simulink model "AGV_IFOC_BLOCKS"  (R2025a)
settings: Solver=ode4  StartTime=0.0  StopTime=t_stop_agv  FixedStep=h_step_agv  RelTol=1e-3
InitFcn:
  | addpath(fileparts(get_param('AGV_IFOC_BLOCKS','FileName'))); bm_drive = 'IFOC'; bm_model = 'AGV_IFOC_BLOCKS'; block_model_params;
values from neighbouring files (symbols this model uses):
  agv_fault_side_default = a.fault_side    [block_model_params.m]
  agv_fault_type_default = a.fault_type    [block_model_params.m]
  Bm = m.B    [block_model_params.m]
  Crr = a.Crr    [block_model_params.m]
  Esw = P.inv.Esw    [block_model_params.m]
  eta_g = a.eta_g    [block_model_params.m]
  flux_mode_default = c.flux_mode    [block_model_params.m]
  G_gear = a.G    [block_model_params.m]
  h_step_agv = 25e-6    (= 2.5e-05)    [block_model_params.m]
  Iref_sw = P.inv.Iref    [block_model_params.m]
  Jm = m.J    [block_model_params.m]
  ke = m.ke    [block_model_params.m]
  kh = m.kh    [block_model_params.m]
  Ki_i = c.Ki_i    [block_model_params.m]
  Ko = c.Ko    [block_model_params.m]
  Kp_i = c.Kp_i    [block_model_params.m]
  Kp_w = c.Kp_w    [block_model_params.m]
  L_look = a.L_look    [block_model_params.m]
  Llr = m.Llr    [block_model_params.m]
  Lls = m.Lls    [block_model_params.m]
  Lm0 = m.Lm0    [block_model_params.m]
  Lm_rated = m.Lm_rated    [block_model_params.m]
  lut_an = P.lut.psi    [block_model_params.m]
  lut_ml = bm_P.lut.psi; end    [block_model_params.m]
  lut_T = P.lut.T(:)'    [block_model_params.m]
  lut_w = P.lut.w(:)'    [block_model_params.m]
  Lx = a.Lx    [block_model_params.m]
  Ly = a.Ly    [block_model_params.m]
  m_payload = a.m_payload    [block_model_params.m]
  m_robot = a.m_robot    [block_model_params.m]
  mlp_b1 = double(bm_M.b1(:))    [block_model_params.m]
  mlp_b2 = double(bm_M.b2)    [block_model_params.m]
  mlp_W1 = double(bm_M.W1)    [block_model_params.m]
  mlp_W2 = double(bm_M.W2(:)')    [block_model_params.m]
  mlp_x_mu = double(bm_M.x_mu(:))    [block_model_params.m]
  mlp_x_sd = double(bm_M.x_sd(:))    [block_model_params.m]
  mlp_y_mu = double(bm_M.y_mu)    [block_model_params.m]
  mlp_y_sd = double(bm_M.y_sd)    [block_model_params.m]
  mras_Ki = c.mras_Ki    [block_model_params.m]
  mras_Kp = c.mras_Kp    [block_model_params.m]
  mras_wc = c.mras_wc    [block_model_params.m]
  NT_agv = max(1, round(Ts/h_step_agv))    [block_model_params.m]
  pp = m.p    [block_model_params.m]
  psi_k = m.psi_k    [block_model_params.m]
  r_wheel = a.r_wheel    [block_model_params.m]
  rce = P.inv.rce    [block_model_params.m]
  Rr = m.Rr    [block_model_params.m]
  Rs = m.Rs    [block_model_params.m]
  s32 = sqrt(3)/2    [block_model_params.m]
  sat_a = m.sat_a    [block_model_params.m]
  sat_b = m.sat_b    [block_model_params.m]
  sat_on = m.sat_on    [block_model_params.m]
  Te_max = c.Te_max    [block_model_params.m]
  Ts = P.ctrl.Ts    [block_log_to_thesis.m]    (also in block_model_params.m = c.Ts)
  twopi = 2*pi    (= 6.28318530718)    [block_model_params.m]
  Vce0 = P.inv.Vce0    [block_model_params.m]
  Vdc = P.inv.Vdc    [block_model_params.m]
  Vref_sw = P.inv.Vref    [block_model_params.m]
  W_track = a.W_track    [block_model_params.m]
(part 1 of 4)
settings Model: Creator=ironman  LastModifiedBy=ironman
settings DataIOCC: SaveOutput=off  SignalLogging=off  SaveTime=off

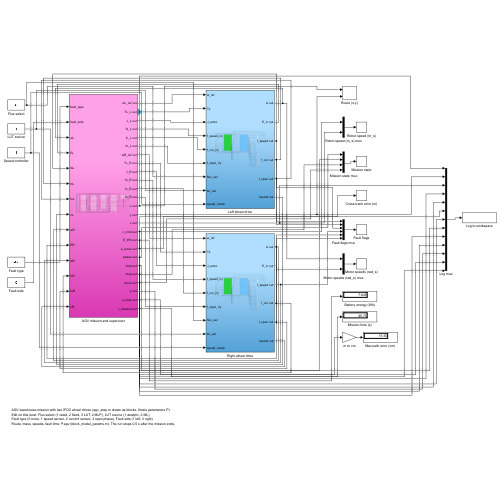
[thumbnail: Simulink's stored preview of the top-level diagram]
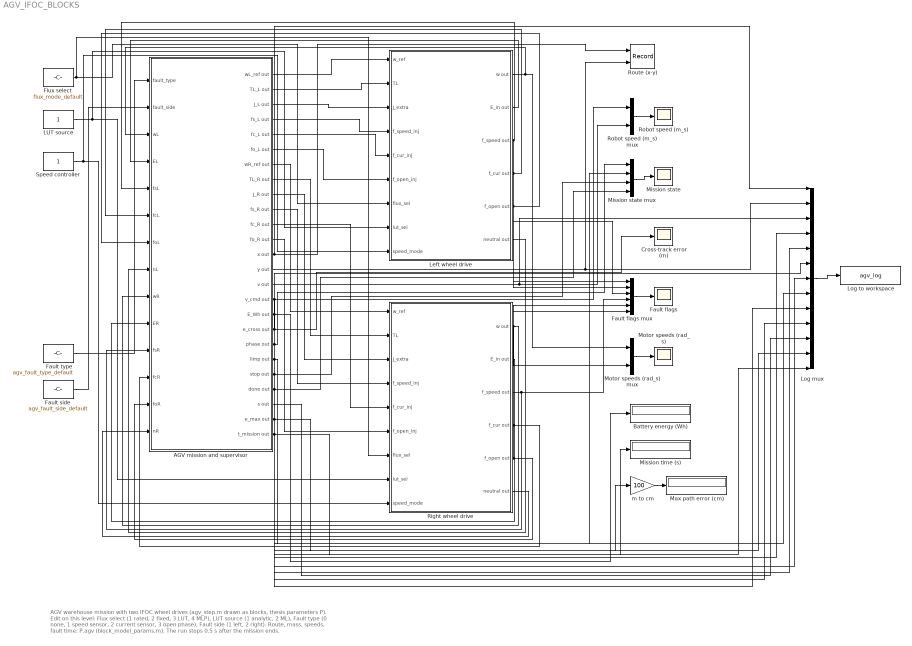
== system AGV_IFOC_BLOCKS ==
  note: AGV warehouse mission with two IFOC wheel drives (agv_step.m drawn as blocks, thesis parameters P).
      | Edit on this level: Flux select (1 rated, 2 fixed, 3 LUT, 4 MLP), LUT source (1 analytic, 2 ML),
      | Fault type (0 none, 1 speed sensor, 2 current sensor, 3 open phase), Fault side (1 left, 2 right).
      | Route, mass, speeds, fault time: P.agv (block_model_params.m). The run stops 0.5 s after the mission ends.
  AGV mission and supervisor : Subsystem
  Battery energy (Wh) : Display
  Cross-track error (m) : Scope
  Fault flags : Scope
  Fault flags mux : Mux  Inputs=6
  Fault side : Constant  Value=agv_fault_side_default
  Fault type : Constant  Value=agv_fault_type_default
  Flux select : Constant  Value=flux_mode_default
  LUT source : Constant
  Left wheel drive : Subsystem
  Log mux : Mux  Inputs=13
  Log to workspace : ToWorkspace  VariableName=agv_log  SaveFormat=Structure With Time  SampleTime=-1
      settings: Decimation=40
  Max path error (cm) : Display
  Mission state : Scope
  Mission state mux : Mux
  Mission time (s) : Display
  Motor speeds (rad_s) : Scope
  Motor speeds (rad_s) mux : Mux  Inputs=2
  Right wheel drive : Subsystem
  Robot speed (m_s) : Scope
  Robot speed (m_s) mux : Mux  Inputs=2
  Route (x-y) : Record  NumPorts=2.0  FileSettingsInternal="{\"entries\":[{\"content\":{\"excelSettings\":{\"content\":{},\"type\":\"Streamout.ExcelSettings\"},\"parquetSettings\":{\"content\":{},\"type\":\"Streamout.ParquetSettings\"}},\"type\":\"Streamout.FileSettingStorage\",\"uuid\":\"\"}],\"packageUris\":[\"http:\\/\\/schema.mathworks.com\\/mf0\\/streamout_blocks\\/R2020a\"],\"version\":\"1.0\"}"  FrameSettings=[0, 0]  Layout=[1 1]  SignalsInternal="{\"entries\":[{\"content\":{\"signals\":[{\"content\":{\"blockPath\":[],\"dimensions\":[1],\"domain\":\"\",\"lineColor\":\"#a2142f\",\"plots\":[ 1 ],\"port\":1,\"sid\":[\"\"],\"signalID\":1,\"signalName\":\"AGV mission and supervisor:13\"},\"type\":\"RecordBlkView.Signal\",\"uuid\":\"\"},{\"content\":{\"blockPath\":[],\"dimensions\":[1],\"domain\":\"\",\"lineColor\":\"#139fff\",\"plots\":[ 1 ],\"port\":2,\"sid\":[\"\"],\"signalID\":2,\"signalName\":\"AGV mission and supervisor:14\"},\"type\":\"RecordBlkView.Signal\",\"uuid\":\"\"}]},\"type\":\"RecordBlkView.InputSignals\",\"uuid\":\"\"}],\"packageUris\":[\"http:\\/\\/schema.mathworks.com\\/mf0\\/streamout_blocks\\/R2020a\"],\"version\":\"1.0\"}"  VisualizationBindings="{\"xyplotplugin\":{\"info\":[{\"series\":[{\"bindingParametersList\":[{\"parameter\":\"X-Axis\",\"signalID\":1,\"signalName\":\"AGV mission and supervisor:13\"},{\"parameter\":\"Y-Axis\",\"signalID\":2,\"signalName\":\"AGV mission and supervisor:14\"}],\"seriesID\":0}],\"subplotID\":1}]}}"  CompatibilityTag=XY
  Speed controller : Constant
  m to cm : Gain  Gain=100
  wires:
  AGV mission and supervisor/1(wL_ref out) -> Left wheel drive/1(w_ref)
  AGV mission and supervisor/2(TL_L out) -> Left wheel drive/2(TL)
  AGV mission and supervisor/3(J_L out) -> Left wheel drive/3(J_extra)
  AGV mission and supervisor/4(fs_L out) -> Left wheel drive/4(f_speed_inj)
  AGV mission and supervisor/5(fc_L out) -> Left wheel drive/5(f_cur_inj)
  AGV mission and supervisor/6(fo_L out) -> Left wheel drive/6(f_open_inj)
  Flux select/1 -> Left wheel drive/7(flux_sel), Right wheel drive/7(flux_sel)
  LUT source/1 -> Left wheel drive/8(lut_sel), Right wheel drive/8(lut_sel)
  Speed controller/1 -> Left wheel drive/9(speed_mode), Right wheel drive/9(speed_mode)
  AGV mission and supervisor/7(wR_ref out) -> Right wheel drive/1(w_ref)
  AGV mission and supervisor/8(TL_R out) -> Right wheel drive/2(TL)
  AGV mission and supervisor/9(J_R out) -> Right wheel drive/3(J_extra)
  AGV mission and supervisor/10(fs_R out) -> Right wheel drive/4(f_speed_inj)
  AGV mission and supervisor/11(fc_R out) -> Right wheel drive/5(f_cur_inj)
  AGV mission and supervisor/12(fo_R out) -> Right wheel drive/6(f_open_inj)
  Fault type/1 -> AGV mission and supervisor/1(fault_type)
  Fault side/1 -> AGV mission and supervisor/2(fault_side)
  Left wheel drive/1(w out) -> AGV mission and supervisor/3(wL), Motor speeds (rad_s) mux/1
  Left wheel drive/2(E_in out) -> AGV mission and supervisor/4(EL)
  Left wheel drive/3(f_speed out) -> AGV mission and supervisor/5(fsL), Fault flags mux/1
  Left wheel drive/4(f_cur out) -> AGV mission and supervisor/6(fcL), Fault flags mux/2
  Left wheel drive/5(f_open out) -> AGV mission and supervisor/7(foL), Fault flags mux/3
  Left wheel drive/6(neutral out) -> AGV mission and supervisor/8(nL)
  Right wheel drive/1(w out) -> AGV mission and supervisor/9(wR), Motor speeds (rad_s) mux/2
  Right wheel drive/2(E_in out) -> AGV mission and supervisor/10(ER)
  Right wheel drive/3(f_speed out) -> AGV mission and supervisor/11(fsR), Fault flags mux/4
  Right wheel drive/4(f_cur out) -> AGV mission and supervisor/12(fcR), Fault flags mux/5
  Right wheel drive/5(f_open out) -> AGV mission and supervisor/13(foR), Fault flags mux/6
  Right wheel drive/6(neutral out) -> AGV mission and supervisor/14(nR)
  AGV mission and supervisor/13(x out) -> Route (x-y)/1, Log mux/1
  AGV mission and supervisor/14(y out) -> Route (x-y)/2, Log mux/2
  AGV mission and supervisor/16(v_cmd out) -> Robot speed (m_s) mux/1, Log mux/4
  AGV mission and supervisor/15(v out) -> Robot speed (m_s) mux/2, Log mux/3
  Robot speed (m_s) mux/1 -> Robot speed (m_s)/1
  AGV mission and supervisor/19(phase out) -> Mission state mux/1, Log mux/7
  AGV mission and supervisor/20(limp out) -> Mission state mux/2, Log mux/8
  AGV mission and supervisor/21(stop out) -> Mission state mux/3, Log mux/9
  AGV mission and supervisor/22(done out) -> Mission state mux/4, Log mux/10
  Mission state mux/1 -> Mission state/1
  AGV mission and supervisor/18(e_cross out) -> Cross-track error (m)/1, Log mux/6
  Fault flags mux/1 -> Fault flags/1
  Motor speeds (rad_s) mux/1 -> Motor speeds (rad_s)/1
  AGV mission and supervisor/17(E_Wh out) -> Battery energy (Wh)/1, Log mux/5
  AGV mission and supervisor/25(t_mission out) -> Mission time (s)/1, Log mux/13
  AGV mission and supervisor/24(e_max out) -> m to cm/1, Log mux/12
  m to cm/1 -> Max path error (cm)/1
  AGV mission and supervisor/23(s out) -> Log mux/11
  Log mux/1 -> Log to workspace/1

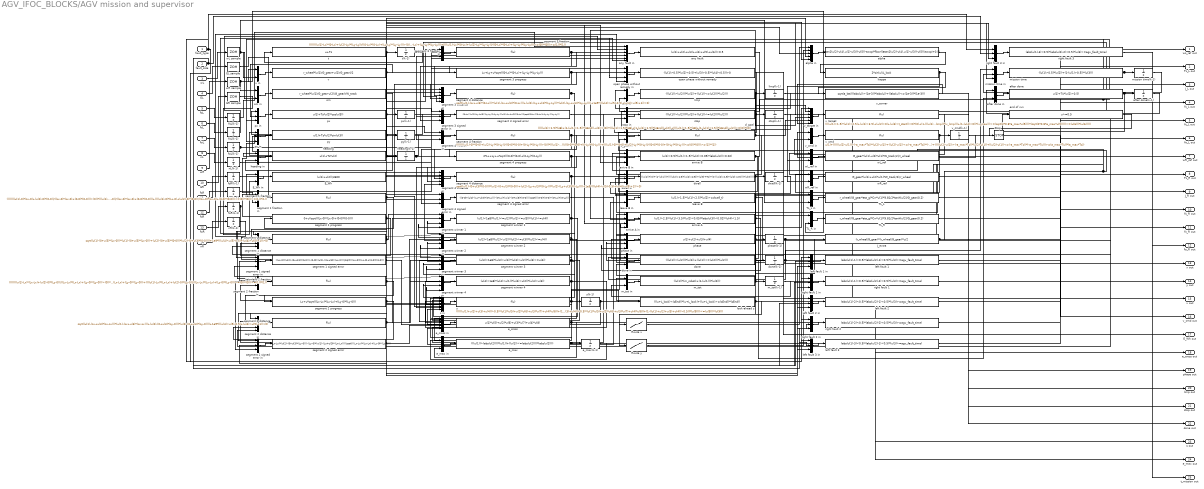
== system AGV_IFOC_BLOCKS/AGV mission and supervisor ==
  fault_type : Inport
  fault_side : Inport  Port=2
  wL : Inport  Port=3
  EL : Inport  Port=4
  fsL : Inport  Port=5
  fcL : Inport  Port=6
  foL : Inport  Port=7
  nL : Inport  Port=8
  wR : Inport  Port=9
  ER : Inport  Port=10
  fsR : Inport  Port=11
  fcR : Inport  Port=12
  foR : Inport  Port=13
  nR : Inport  Port=14
  EL sample : ZeroOrderHold  SampleTime=Ts
  ER sample : ZeroOrderHold  SampleTime=Ts
  E_Wh : Fcn  Expr=(u(1)+u(2))/3600
  E_Wh in : Mux  Inputs=2
  J_extra : Fcn  Expr=(r_wheel/G_gear)*(r_wheel/G_gear)*u/2
  Route x : Lookup_n-D  NumberOfTableDimensions=1  BreakpointsForDimension1=[0 Lx Lx+Ly 2*Lx+Ly 2*(Lx+Ly)]  Table=[0 Lx Lx 0 0]  ExtrapMethod=Clip  InternalRulePriority=Speed  RndMeth=Simplest
  Route y : Lookup_n-D  NumberOfTableDimensions=1  BreakpointsForDimension1=[0 Lx Lx+Ly 2*Lx+Ly 2*(Lx+Ly)]  Table=[0 0 Ly Ly 0]  ExtrapMethod=Clip  InternalRulePriority=Speed  RndMeth=Simplest
  Stop : Stop
  TL_L : Fcn  Expr=r_wheel/(G_gear*eta_g)*Crr*u(1)*9.81/2*tanh(u(2)/G_gear/0.2)
  TL_L in : Mux  Inputs=2
  TL_R : Fcn  Expr=r_wheel/(G_gear*eta_g)*Crr*u(1)*9.81/2*tanh(u(2)/G_gear/0.2)
  TL_R in : Mux  Inputs=2
  after done : Fcn  Expr=u(1)+Ts*(u(2)>0.5)
  after done in : Mux  Inputs=2
  after done(k-1) : UnitDelay  SampleTime=Ts  HasFrameUpgradeWarning=on
  alpha : Fcn  Expr=(atan2(u(2)-u(4),u(1)-u(3))-u(5))-twopi*floor((atan2(u(2)-u(4),u(1)-u(3))-u(5))/twopi+0.5)
  alpha in : Mux  Inputs=5
  any fault : Fcn  Expr=(u(1)+u(2)+u(3)+u(4)+u(5)+u(6))>0.5
  any fault in : Mux  Inputs=6
  arrive A : Fcn  Expr=(u(1)>2.5)*(u(1)<3.5)*(u(2)<0.05)*(abs(u(3))<0.02)*(u(4)<1.5)
  arrive A in : Mux
  arrive B : Fcn  Expr=(u(1)>0.5)*(u(1)<1.5)*(u(2)<0.05)*(abs(u(3))<0.02)
  arrive B in : Mux  Inputs=3
  d_goal : Fcn  Expr=(((((u(1)<1.5)*(sB)+(1-(u(1)<1.5))*(sEnd))-u(2))>(0))*(((u(1)<1.5)*(sB)+(1-(u(1)<1.5))*(sEnd))-u(2))+((((u(1)<1.5)*(sB)+(1-(u(1)<1.5))*(sEnd))-u(2))<=(0))*(0))
  d_goal in : Mux  Inputs=2
  done : Fcn  Expr=(((u(1))>(u(2)))*(u(1))+((u(1))<=(u(2)))*(u(2)))
  done in : Mux  Inputs=2
  done(k-1) : UnitDelay  SampleTime=Ts  HasFrameUpgradeWarning=on
  dwell : Fcn  Expr=((u(1))*(0)+(1-(u(1)))*((((u(2)>1.5)*(u(2)<2.5))*(u(3)+Ts)+(1-((u(2)>1.5)*(u(2)<2.5)))*(u(3)))))
  dwell in : Mux  Inputs=3
  dwell(k-1) : UnitDelay  SampleTime=Ts  HasFrameUpgradeWarning=on
  e_cross : Fcn  Expr=u(1)*u(5)+u(2)*u(6)+u(3)*u(7)+u(4)*u(8)
  e_cross in : Mux  Inputs=8
  e_max : Fcn  Expr=(((u(1))>(abs(u(2))))*(u(1))+((u(1))<=(abs(u(2))))*(abs(u(2))))
  e_max in : Mux  Inputs=2
  e_max(k-1) : UnitDelay  SampleTime=Ts  HasFrameUpgradeWarning=on
  end of run : Fcn  Expr=u>=0.5
  fcL(k-1) : UnitDelay  SampleTime=Ts  HasFrameUpgradeWarning=on
  fcR(k-1) : UnitDelay  SampleTime=Ts  HasFrameUpgradeWarning=on
  foL(k-1) : UnitDelay  SampleTime=Ts  HasFrameUpgradeWarning=on
  foR(k-1) : UnitDelay  SampleTime=Ts  HasFrameUpgradeWarning=on
  fsL(k-1) : UnitDelay  SampleTime=Ts  HasFrameUpgradeWarning=on
  fsR(k-1) : UnitDelay  SampleTime=Ts  HasFrameUpgradeWarning=on
  heading : Fcn  Expr=u(1)+Ts*u(2)
  heading in : Mux  Inputs=2
  heading(k-1) : UnitDelay  SampleTime=Ts  HasFrameUpgradeWarning=on
  kappa : Fcn  Expr=2*sin(u)/L_look
  leave B : Fcn  Expr=(u(1)>1.5)*(u(1)<2.5)*(u(2)>=dwell_t)
  leave B in : Mux  Inputs=2
  left fault 1 : Fcn  Expr=(abs(u(1)-1)<0.5)*(abs(u(2)-1)<0.5)*(u(3)>=agv_fault_time)
  left fault 1 in : Mux  Inputs=3
  left fault 2 : Fcn  Expr=(abs(u(1)-2)<0.5)*(abs(u(2)-1)<0.5)*(u(3)>=agv_fault_time)
  left fault 2 in : Mux  Inputs=3
  left fault 3 : Fcn  Expr=(abs(u(1)-3)<0.5)*(abs(u(2)-1)<0.5)*(u(3)>=agv_fault_time)
  left fault 3 in : Mux  Inputs=3
  limp : Fcn  Expr=(((u(1))>(u(2)))*(u(1))+((u(1))<=(u(2)))*(u(2)))
  limp in : Mux  Inputs=2
  limp(k-1) : UnitDelay  SampleTime=Ts  HasFrameUpgradeWarning=on
  look-ahead s : Fcn  Expr=(((u+L_look)<(sEnd))*(u+L_look)+((u+L_look)>=(sEnd))*(sEnd))
  m_tot : Fcn  Expr=((u(1))*(m_robot)+(1-(u(1)))*(u(2)))
  m_tot in : Mux  Inputs=2
  m_tot(k-1) : UnitDelay  InitialCondition=m_robot+m_payload  SampleTime=Ts  HasFrameUpgradeWarning=on
  mission time : Fcn  Expr=((u(1)>0.5)*(u(2))+(1-(u(1)>0.5))*(u(3)))
  mission time in : Mux  Inputs=3
  mission time(k-1) : UnitDelay  SampleTime=Ts  HasFrameUpgradeWarning=on
  nL(k-1) : UnitDelay  SampleTime=Ts  HasFrameUpgradeWarning=on
  nR(k-1) : UnitDelay  SampleTime=Ts  HasFrameUpgradeWarning=on
  om : Fcn  Expr=r_wheel*(u(1)/G_gear-u(2)/G_gear)/W_track
  om in : Mux  Inputs=2
  open phase without remedy : Fcn  Expr=((u(1)>0.5)*(u(2)<0.5)+(u(3)>0.5)*(u(4)<0.5))>0
  open phase without remedy in : Mux
  phase : Fcn  Expr=u(1)+u(2)+u(3)+u(4)
  phase in : Mux
  phase(k-1) : UnitDelay  InitialCondition=1  SampleTime=Ts  HasFrameUpgradeWarning=on
  px : Fcn  Expr=u(1)+Ts*u(2)*cos(u(3))
  px in : Mux  Inputs=3
  px(k-1) : UnitDelay  SampleTime=Ts  HasFrameUpgradeWarning=on
  py : Fcn  Expr=u(1)+Ts*u(2)*sin(u(3))
  py in : Mux  Inputs=3
  py(k-1) : UnitDelay  SampleTime=Ts  HasFrameUpgradeWarning=on
  right fault 1 : Fcn  Expr=(abs(u(1)-1)<0.5)*(abs(u(2)-2)<0.5)*(u(3)>=agv_fault_time)
  right fault 1 in : Mux  Inputs=3
  right fault 2 : Fcn  Expr=(abs(u(1)-2)<0.5)*(abs(u(2)-2)<0.5)*(u(3)>=agv_fault_time)
  right fault 2 in : Mux  Inputs=3
  right fault 3 : Fcn  Expr=(abs(u(1)-3)<0.5)*(abs(u(2)-2)<0.5)*(u(3)>=agv_fault_time)
  right fault 3 in : Mux  Inputs=3
  s : Fcn  Expr=((((((u(1)+u(2)+u(3)+u(4))>0.5)*(u(1)*u(5)+u(2)*u(6)+u(3)*u(7)+u(4)*u(8))+(1-((u(1)+u(2)+u(3)+u(4))>0.5))*(u(9))))>(u(9)))*((((u(1)+u(2)+u(3)+u(4))>0.5)*(u(1)*u(5)+u(2)*u(6)+u(3)*u(7)+u(4)*u(8))+(1-((u(1)+u(2)+u(3)+u(4))>0.5))*(u(9))))+(((((u(1)+u(2)+u(3)+u(4))>0.5)*(u(1)*u(5)+u(2)*u(6)+u(3)*u(7)+u(4)*u(8))+(1-((u(1)+u(2)+u(3)+u(4))>0.5))*(u(9))))<=(u(9)))*(u(9)))
  s in : Mux  Inputs=9
  s(k-1) : UnitDelay  SampleTime=Ts  HasFrameUpgradeWarning=on
  segment 1 distance : Fcn  Expr=sqrt((u(1)-(0+u(3)*(Lx-0)))*(u(1)-(0+u(3)*(Lx-0)))+(u(2)-(0+u(3)*(0-0)))*(u(2)-(0+u(3)*(0-0))))+1e9*(((u(4)<u(5)-0.5)+(u(4)>u(5)+1))>0)
  segment 1 distance in : Mux  Inputs=5
  segment 1 fraction : Fcn  Expr=((((((((u(1)-0)*(Lx-0)+(u(2)-0)*(0-0))/((Lx-0)*(Lx-0)+(0-0)*(0-0)))>(0))*(((u(1)-0)*(Lx-0)+(u(2)-0)*(0-0))/((Lx-0)*(Lx-0)+(0-0)*(0-0)))+((((u(1)-0)*(Lx-0)+(u(2)-0)*(0-0))/((Lx-0)*(Lx-0)+(0-0)*(0-0)))<=(0))*(0)))<(1))*((((((u(1)-0)*(Lx-0)+(u(2)-0)*(0-0))/((Lx-0)*(Lx-0)+(0-0)*(0-0)))>(0))*(((u(1)-0)*(Lx-0)+(u(2)-0)*(0-0))/((Lx-0)*(Lx-0)+(0-0)*(0-0)))+((((u(1)-0)*(Lx-0)+(u(2)-0)*(0-0))/((Lx-0)*(Lx-0)+(0-0)*(0-0)))<=(0))*(0)))+(((((((u(1)-0)*(Lx-0)+(u(2)-0)*(0-0))/((Lx-0)*(Lx-0)+(0-0)*(0-0)))>(0))*(((u(1)-0)*(Lx-0)+(u(2)-0)*(0-0))/((Lx-0)*(Lx-0)+(0-0)*(0-0)))+((((u(1)-0)*(Lx-0)+(u(2)-0)*(0-0))/((Lx-0)*(Lx-0)+(0-0)*(0-0)))<=(0))*(0)))>=(1))*(1))
  segment 1 fraction in : Mux  Inputs=2
  segment 1 progress : Fcn  Expr=0+u*sqrt(((Lx-0)*(Lx-0)+(0-0)*(0-0)))
  segment 1 signed error : Fcn  Expr=((Lx-0)*(u(2)-(0+u(3)*(0-0)))-(0-0)*(u(1)-(0+u(3)*(Lx-0))))/sqrt(((Lx-0)*(Lx-0)+(0-0)*(0-0)))
  segment 1 signed error in : Mux  Inputs=3
  segment 2 distance : Fcn  Expr=sqrt((u(1)-(Lx+u(3)*(Lx-Lx)))*(u(1)-(Lx+u(3)*(Lx-Lx)))+(u(2)-(0+u(3)*(Ly-0)))*(u(2)-(0+u(3)*(Ly-0))))+1e9*(((u(4)<u(5)-0.5)+(u(4)>u(5)+1))>0)
  segment 2 distance in : Mux  Inputs=5
  segment 2 fraction : Fcn  Expr=((((((((u(1)-Lx)*(Lx-Lx)+(u(2)-0)*(Ly-0))/((Lx-Lx)*(Lx-Lx)+(Ly-0)*(Ly-0)))>(0))*(((u(1)-Lx)*(Lx-Lx)+(u(2)-0)*(Ly-0))/((Lx-Lx)*(Lx-Lx)+(Ly-0)*(Ly-0)))+((((u(1)-Lx)*(Lx-Lx)+(u(2)-0)*(Ly-0))/((Lx-Lx)*(Lx-Lx)+(Ly-0)*(Ly-0)))<=(0))*(0)))<(1))*((((((u(1)-Lx)*(Lx-Lx)+(u(2)-0)*(Ly-0))/((Lx-Lx)*(Lx-Lx)+(Ly-0)*(Ly-0)))>(0))*(((u(1)-Lx)*(Lx-Lx)+(u(2)-0)*(Ly-0))/((Lx-Lx)*(Lx-Lx)+(Ly-0)*(Ly-0)))+((((u(1)-Lx)*(Lx-Lx)+(u(2)-0)*(Ly-0))/((Lx-Lx)*(Lx-Lx)+(Ly-0)*(Ly-0)))<=(0))*(0)))+(((((((u(1)-Lx)*(Lx-Lx)+(u(2)-0)*(Ly-0))/((Lx-Lx)*(Lx-Lx)+(Ly-0)*(Ly-0)))>(0))*(((u(1)-Lx)*(Lx-Lx)+(u(2)-0)*(Ly-0))/((Lx-Lx)*(Lx-Lx)+(Ly-0)*(Ly-0)))+((((u(1)-Lx)*(Lx-Lx)+(u(2)-0)*(Ly-0))/((Lx-Lx)*(Lx-Lx)+(Ly-0)*(Ly-0)))<=(0))*(0)))>=(1))*(1))
  segment 2 fraction in : Mux  Inputs=2
  segment 2 progress : Fcn  Expr=Lx+u*sqrt(((Lx-Lx)*(Lx-Lx)+(Ly-0)*(Ly-0)))
  segment 2 signed error : Fcn  Expr=((Lx-Lx)*(u(2)-(0+u(3)*(Ly-0)))-(Ly-0)*(u(1)-(Lx+u(3)*(Lx-Lx))))/sqrt(((Lx-Lx)*(Lx-Lx)+(Ly-0)*(Ly-0)))
  segment 2 signed error in : Mux  Inputs=3
  segment 3 distance : Fcn  Expr=sqrt((u(1)-(Lx+u(3)*(0-Lx)))*(u(1)-(Lx+u(3)*(0-Lx)))+(u(2)-(Ly+u(3)*(Ly-Ly)))*(u(2)-(Ly+u(3)*(Ly-Ly))))+1e9*(((u(4)<u(5)-0.5)+(u(4)>u(5)+1))>0)
  segment 3 distance in : Mux  Inputs=5
  segment 3 fraction : Fcn  Expr=((((((((u(1)-Lx)*(0-Lx)+(u(2)-Ly)*(Ly-Ly))/((0-Lx)*(0-Lx)+(Ly-Ly)*(Ly-Ly)))>(0))*(((u(1)-Lx)*(0-Lx)+(u(2)-Ly)*(Ly-Ly))/((0-Lx)*(0-Lx)+(Ly-Ly)*(Ly-Ly)))+((((u(1)-Lx)*(0-Lx)+(u(2)-Ly)*(Ly-Ly))/((0-Lx)*(0-Lx)+(Ly-Ly)*(Ly-Ly)))<=(0))*(0)))<(1))*((((((u(1)-Lx)*(0-Lx)+(u(2)-Ly)*(Ly-Ly))/((0-Lx)*(0-Lx)+(Ly-Ly)*(Ly-Ly)))>(0))*(((u(1)-Lx)*(0-Lx)+(u(2)-Ly)*(Ly-Ly))/((0-Lx)*(0-Lx)+(Ly-Ly)*(Ly-Ly)))+((((u(1)-Lx)*(0-Lx)+(u(2)-Ly)*(Ly-Ly))/((0-Lx)*(0-Lx)+(Ly-Ly)*(Ly-Ly)))<=(0))*(0)))+(((((((u(1)-Lx)*(0-Lx)+(u(2)-Ly)*(Ly-Ly))/((0-Lx)*(0-Lx)+(Ly-Ly)*(Ly-Ly)))>(0))*(((u(1)-Lx)*(0-Lx)+(u(2)-Ly)*(Ly-Ly))/((0-Lx)*(0-Lx)+(Ly-Ly)*(Ly-Ly)))+((((u(1)-Lx)*(0-Lx)+(u(2)-Ly)*(Ly-Ly))/((0-Lx)*(0-Lx)+(Ly-Ly)*(Ly-Ly)))<=(0))*(0)))>=(1))*(1))
  segment 3 fraction in : Mux  Inputs=2
  segment 3 progress : Fcn  Expr=Lx+Ly+u*sqrt(((0-Lx)*(0-Lx)+(Ly-Ly)*(Ly-Ly)))
  segment 3 signed error : Fcn  Expr=((0-Lx)*(u(2)-(Ly+u(3)*(Ly-Ly)))-(Ly-Ly)*(u(1)-(Lx+u(3)*(0-Lx))))/sqrt(((0-Lx)*(0-Lx)+(Ly-Ly)*(Ly-Ly)))
  segment 3 signed error in : Mux  Inputs=3
  segment 4 distance : Fcn  Expr=sqrt((u(1)-(0+u(3)*(0-0)))*(u(1)-(0+u(3)*(0-0)))+(u(2)-(Ly+u(3)*(0-Ly)))*(u(2)-(Ly+u(3)*(0-Ly))))+1e9*(((u(4)<u(5)-0.5)+(u(4)>u(5)+1))>0)
  segment 4 distance in : Mux  Inputs=5
  segment 4 fraction : Fcn  Expr=((((((((u(1)-0)*(0-0)+(u(2)-Ly)*(0-Ly))/((0-0)*(0-0)+(0-Ly)*(0-Ly)))>(0))*(((u(1)-0)*(0-0)+(u(2)-Ly)*(0-Ly))/((0-0)*(0-0)+(0-Ly)*(0-Ly)))+((((u(1)-0)*(0-0)+(u(2)-Ly)*(0-Ly))/((0-0)*(0-0)+(0-Ly)*(0-Ly)))<=(0))*(0)))<(1))*((((((u(1)-0)*(0-0)+(u(2)-Ly)*(0-Ly))/((0-0)*(0-0)+(0-Ly)*(0-Ly)))>(0))*(((u(1)-0)*(0-0)+(u(2)-Ly)*(0-Ly))/((0-0)*(0-0)+(0-Ly)*(0-Ly)))+((((u(1)-0)*(0-0)+(u(2)-Ly)*(0-Ly))/((0-0)*(0-0)+(0-Ly)*(0-Ly)))<=(0))*(0)))+(((((((u(1)-0)*(0-0)+(u(2)-Ly)*(0-Ly))/((0-0)*(0-0)+(0-Ly)*(0-Ly)))>(0))*(((u(1)-0)*(0-0)+(u(2)-Ly)*(0-Ly))/((0-0)*(0-0)+(0-Ly)*(0-Ly)))+((((u(1)-0)*(0-0)+(u(2)-Ly)*(0-Ly))/((0-0)*(0-0)+(0-Ly)*(0-Ly)))<=(0))*(0)))>=(1))*(1))
  segment 4 fraction in : Mux  Inputs=2
  segment 4 progress : Fcn  Expr=2*Lx+Ly+u*sqrt(((0-0)*(0-0)+(0-Ly)*(0-Ly)))
  segment 4 signed error : Fcn  Expr=((0-0)*(u(2)-(Ly+u(3)*(0-Ly)))-(0-Ly)*(u(1)-(0+u(3)*(0-0))))/sqrt(((0-0)*(0-0)+(0-Ly)*(0-Ly)))
  segment 4 signed error in : Mux  Inputs=3
  segment winner 1 : Fcn  Expr=(u(1)<1e8)*(u(1)<=u(2))*(u(1)<=u(3))*(u(1)<=u(4))
  segment winner 1 in : Mux
  segment winner 2 : Fcn  Expr=(u(2)<1e8)*(u(2)<u(1))*(u(2)<=u(3))*(u(2)<=u(4))
  segment winner 2 in : Mux
  segment winner 3 : Fcn  Expr=(u(3)<1e8)*(u(3)<u(1))*(u(3)<u(2))*(u(3)<=u(4))
  segment winner 3 in : Mux
  segment winner 4 : Fcn  Expr=(u(4)<1e8)*(u(4)<u(1))*(u(4)<u(2))*(u(4)<u(3))
  segment winner 4 in : Mux
  stop : Fcn  Expr=(((u(1))>(u(2)))*(u(1))+((u(1))<=(u(2)))*(u(2)))
  stop in : Mux  Inputs=2
  stop(k-1) : UnitDelay  SampleTime=Ts  HasFrameUpgradeWarning=on
  t : Fcn  Expr=u+Ts
  t(k-1) : UnitDelay  SampleTime=Ts  HasFrameUpgradeWarning=on
  v : Fcn  Expr=r_wheel*(u(1)/G_gear+u(2)/G_gear)/2
  v in : Mux  Inputs=2
  v_cmd : Fcn  Expr=u(1)+((((((u(2)-u(1))>(-a_max*Ts))*(u(2)-u(1))+((u(2)-u(1))<=(-a_max*Ts))*(-a_max*Ts)))<(a_max*Ts))*((((u(2)-u(1))>(-a_max*Ts))*(u(2)-u(1))+((u(2)-u(1))<=(-a_max*Ts))*(-a_max*Ts)))+(((((u(2)-u(1))>(-a_max*Ts))*(u(2)-u(1))+((u(2)-u(1))<=(-a_max*Ts))*(-a_max*Ts)))>=(a_max*Ts))*(a_max*Ts))
  v_cmd in : Mux  Inputs=2
  v_cmd(k-1) : UnitDelay  SampleTime=Ts  HasFrameUpgradeWarning=on
  v_corner : Fcn  Expr=sqrt(a_lat/(((abs(u))>(1e-3))*(abs(u))+((abs(u))<=(1e-3))*(1e-3)))
  v_target : Fcn  Expr=((((u(1)>1.5)*(u(1)<2.5)+(u(1)>3.5)+(u(2)>0)+(u(3)<t_start))>0)*(0)+(1-(((u(1)>1.5)*(u(1)<2.5)+(u(1)>3.5)+(u(2)>0)+(u(3)<t_start))>0))*(((((((((u(4)>0)*((((v_max)<(v_limp))*(v_max)+((v_max)>=(v_limp))*(v_limp)))+(1-(u(4)>0))*(v_max)))<(sqrt(2*0.8*a_max*u(5))))*(((u(4)>0)*((((v_max)<(v_limp))*(v_max)+((v_max)>=(v_limp))*(v_limp)))+(1-(u(4)>0))*(v_max)))+((((u(4)>0)*((((v_max)<(v_limp))*(v_max)+((v_max)>=(v_limp))*(v_limp)))+(1-(u(4)>0))*(v_max)))>=(sqrt(2*0.8*a_max*u(5))))*(sqrt(2*0.8*a_max*u(5)))))<(u(6)))*((((((u(4)>0)*((((v_max)<(v_limp))*(v_max)+((v_max)>=(v_limp))*(v_limp)))+(1-(u(4)>0))*(v_max)))<(sqrt(2*0.8*a_max*u(5))))*(((u(4)>0)*((((v_max)<(v_limp))*(v_max)+((v_max)>=(v_limp))*(v_limp)))+(1-(u(4)>0))*(v_max)))+((((u(4)>0)*((((v_max)<(v_limp))*(v_max)+((v_max)>=(v_limp))*(v_limp)))+(1-(u(4)>0))*(v_max)))>=(sqrt(2*0.8*a_max*u(5))))*(sqrt(2*0.8*a_max*u(5)))))+(((((((u(4)>0)*((((v_max)<(v_limp))*(v_max)+((v_max)>=(v_limp))*(v_limp)))+(1-(u(4)>0))*(v_max)))<(sqrt(2*0.8*a_max*u(5))))*(((u(4)>0)*((((v_max)<(v_limp))*(v_max)+((v_max)>=(v_limp))*(v_limp)))+(1-(u(4)>0))*(v_max)))+((((u(4)>0)*((((v_max)<(v_limp))*(v_max)+((v_max)>=(v_limp))*(v_limp)))+(1-(u(4)>0))*(v_max)))>=(sqrt(2*0.8*a_max*u(5))))*(sqrt(2*0.8*a_max*u(5)))))>=(u(6)))*(u(6)))))
  v_target in : Mux  Inputs=6
  wL sample : ZeroOrderHold  SampleTime=Ts
  wL_ref : Fcn  Expr=G_gear*(u(1)-u(2)*u(1)*W_track/2)/r_wheel
  wL_ref in : Mux  Inputs=2
  wR sample : ZeroOrderHold  SampleTime=Ts
  wR_ref : Fcn  Expr=G_gear*(u(1)+u(2)*u(1)*W_track/2)/r_wheel
  wR_ref in : Mux  Inputs=2
  wL_ref out : Outport
  TL_L out : Outport  Port=2
  J_L out : Outport  Port=3
  fs_L out : Outport  Port=4
  fc_L out : Outport  Port=5
  fo_L out : Outport  Port=6
  wR_ref out : Outport  Port=7
  TL_R out : Outport  Port=8
  J_R out : Outport  Port=9
  fs_R out : Outport  Port=10
  fc_R out : Outport  Port=11
  fo_R out : Outport  Port=12
  x out : Outport  Port=13
  y out : Outport  Port=14
  v out : Outport  Port=15
  v_cmd out : Outport  Port=16
  E_Wh out : Outport  Port=17
  e_cross out : Outport  Port=18
  phase out : Outport  Port=19
  limp out : Outport  Port=20
  stop out : Outport  Port=21
  done out : Outport  Port=22
  s out : Outport  Port=23
  e_max out : Outport  Port=24
  t_mission out : Outport  Port=25
  wires:
  wL/1 -> wL sample/1
  EL/1 -> EL sample/1
  wR/1 -> wR sample/1
  ER/1 -> ER sample/1
  fsL/1 -> fsL(k-1)/1
  fcL/1 -> fcL(k-1)/1
  foL/1 -> foL(k-1)/1
  nL/1 -> nL(k-1)/1
  fsR/1 -> fsR(k-1)/1
  fcR/1 -> fcR(k-1)/1
  foR/1 -> foR(k-1)/1
  nR/1 -> nR(k-1)/1
  t(k-1)/1 -> t/1
  t/1 -> t(k-1)/1, v_target in/3, left fault 1 in/3, right fault 1 in/3, left fault 2 in/3, right fault 2 in/3, left fault 3 in/3, right fault 3 in/3, mission time in/3
  wR sample/1 -> v in/1, om in/1, TL_R in/2
  wL sample/1 -> v in/2, om in/2, TL_L in/2
  v in/1 -> v/1
  om in/1 -> om/1
  px(k-1)/1 -> px in/1
  v/1 -> px in/2, py in/2, arrive B in/3, arrive A in/3, v out/1
  heading(k-1)/1 -> px in/3, py in/3, heading in/1
  px in/1 -> px/1
  px/1 -> px(k-1)/1, segment 1 fraction in/1, segment 1 distance in/1, segment 1 signed error in/1, segment 2 fraction in/1, segment 2 distance in/1, segment 2 signed error in/1, segment 3 fraction in/1, segment 3 distance in/1, segment 3 signed error in/1, segment 4 fraction in/1, segment 4 distance in/1, segment 4 signed error in/1, alpha in/3, x out/1
  py(k-1)/1 -> py in/1
  py in/1 -> py/1
  py/1 -> py(k-1)/1, segment 1 fraction in/2, segment 1 distance in/2, segment 1 signed error in/2, segment 2 fraction in/2, segment 2 distance in/2, segment 2 signed error in/2, segment 3 fraction in/2, segment 3 distance in/2, segment 3 signed error in/2, segment 4 fraction in/2, segment 4 distance in/2, segment 4 signed error in/2, alpha in/4, y out/1
  om/1 -> heading in/2
  heading in/1 -> heading/1
  heading/1 -> heading(k-1)/1, alpha in/5
  EL sample/1 -> E_Wh in/1
  ER sample/1 -> E_Wh in/2
  E_Wh in/1 -> E_Wh/1
  segment 1 fraction in/1 -> segment 1 fraction/1
  segment 1 fraction/1 -> segment 1 progress/1, segment 1 distance in/3, segment 1 signed error in/3
  segment 1 progress/1 -> segment 1 distance in/4, s in/5
  s(k-1)/1 -> segment 1 distance in/5, segment 2 distance in/5, segment 3 distance in/5, segment 4 distance in/5, s in/9
  segment 1 distance in/1 -> segment 1 distance/1
  segment 1 signed error in/1 -> segment 1 signed error/1
  segment 2 fraction in/1 -> segment 2 fraction/1
  segment 2 fraction/1 -> segment 2 progress/1, segment 2 distance in/3, segment 2 signed error in/3
  segment 2 progress/1 -> segment 2 distance in/4, s in/6
  segment 2 distance in/1 -> segment 2 distance/1
  segment 2 signed error in/1 -> segment 2 signed error/1
  segment 3 fraction in/1 -> segment 3 fraction/1
  segment 3 fraction/1 -> segment 3 progress/1, segment 3 distance in/3, segment 3 signed error in/3
  segment 3 progress/1 -> segment 3 distance in/4, s in/7
  segment 3 distance in/1 -> segment 3 distance/1
  segment 3 signed error in/1 -> segment 3 signed error/1
  segment 4 fraction in/1 -> segment 4 fraction/1
  segment 4 fraction/1 -> segment 4 progress/1, segment 4 distance in/3, segment 4 signed error in/3
  segment 4 progress/1 -> segment 4 distance in/4, s in/8
  segment 4 distance in/1 -> segment 4 distance/1
  segment 4 signed error in/1 -> segment 4 signed error/1
  segment 1 distance/1 -> segment winner 1 in/1, segment winner 2 in/1, segment winner 3 in/1, segment winner 4 in/1
  segment 2 distance/1 -> segment winner 1 in/2, segment winner 2 in/2, segment winner 3 in/2, segment winner 4 in/2
  segment 3 distance/1 -> segment winner 1 in/3, segment winner 2 in/3, segment winner 3 in/3, segment winner 4 in/3
  segment 4 distance/1 -> segment winner 1 in/4, segment winner 2 in/4, segment winner 3 in/4, segment winner 4 in/4
  segment winner 1 in/1 -> segment winner 1/1
  segment winner 2 in/1 -> segment winner 2/1
  segment winner 3 in/1 -> segment winner 3/1
  segment winner 4 in/1 -> segment winner 4/1
  segment winner 1/1 -> s in/1, e_cross in/1
  segment winner 2/1 -> s in/2, e_cross in/2
  segment winner 3/1 -> s in/3, e_cross in/3
  segment winner 4/1 -> s in/4, e_cross in/4
  s in/1 -> s/1
  s/1 -> s(k-1)/1, d_goal in/2, look-ahead s/1, s out/1
  segment 1 signed error/1 -> e_cross in/5
  segment 2 signed error/1 -> e_cross in/6
  segment 3 signed error/1 -> e_cross in/7
  segment 4 signed error/1 -> e_cross in/8
  e_cross in/1 -> e_cross/1
  e_max(k-1)/1 -> e_max in/1
  e_cross/1 -> e_max in/2, e_cross out/1
  e_max in/1 -> e_max/1
  e_max/1 -> e_max(k-1)/1, e_max out/1
  fsL(k-1)/1 -> any fault in/1
  fcL(k-1)/1 -> any fault in/2
  foL(k-1)/1 -> any fault in/3, open phase without remedy in/1
  fsR(k-1)/1 -> any fault in/4
  fcR(k-1)/1 -> any fault in/5
  foR(k-1)/1 -> any fault in/6, open phase without remedy in/3
  any fault in/1 -> any fault/1
  nL(k-1)/1 -> open phase without remedy in/2
  nR(k-1)/1 -> open phase without remedy in/4
  open phase without remedy in/1 -> open phase without remedy/1
  limp(k-1)/1 -> limp in/1
  any fault/1 -> limp in/2
  limp in/1 -> limp/1
  limp/1 -> limp(k-1)/1, v_target in/4, limp out/1
  stop(k-1)/1 -> stop in/1
  open phase without remedy/1 -> stop in/2
  stop in/1 -> stop/1
  stop/1 -> stop(k-1)/1, v_target in/2, stop out/1
  phase(k-1)/1 -> d_goal in/1, arrive B in/1, dwell in/2, leave B in/1, arrive A in/1, phase in/1
  d_goal in/1 -> d_goal/1
  d_goal/1 -> arrive B in/2, arrive A in/2, v_target in/5
  arrive B in/1 -> arrive B/1
  arrive B/1 -> dwell in/1, phase in/2
  dwell(k-1)/1 -> dwell in/3
  dwell in/1 -> dwell/1
  dwell/1 -> dwell(k-1)/1, leave B in/2
  leave B in/1 -> leave B/1
  done(k-1)/1 -> arrive A in/4, done in/1, mission time in/1
  arrive A in/1 -> arrive A/1
  leave B/1 -> phase in/3, m_tot in/1
  arrive A/1 -> phase in/4, done in/2
  phase in/1 -> phase/1
  phase/1 -> phase(k-1)/1, v_target in/1, phase out/1
  done in/1 -> done/1
  done/1 -> done(k-1)/1, after done in/2, done out/1
  m_tot(k-1)/1 -> m_tot in/2
  m_tot in/1 -> m_tot/1
  m_tot/1 -> m_tot(k-1)/1, TL_L in/1, TL_R in/1, J_extra/1
  look-ahead s/1 -> Route x/1, Route y/1
  Route x/1 -> alpha in/1
  Route y/1 -> alpha in/2
  alpha in/1 -> alpha/1
  alpha/1 -> kappa/1
  kappa/1 -> v_corner/1, wL_ref in/2, wR_ref in/2
  v_corner/1 -> v_target in/6
  v_target in/1 -> v_target/1
  v_cmd(k-1)/1 -> v_cmd in/1
  v_target/1 -> v_cmd in/2
  v_cmd in/1 -> v_cmd/1
  v_cmd/1 -> v_cmd(k-1)/1, wL_ref in/1, wR_ref in/1, v_cmd out/1
  wL_ref in/1 -> wL_ref/1
  wR_ref in/1 -> wR_ref/1
  TL_L in/1 -> TL_L/1
  TL_R in/1 -> TL_R/1
  fault_type/1 -> left fault 1 in/1, right fault 1 in/1, left fault 2 in/1, right fault 2 in/1, left fault 3 in/1, right fault 3 in/1
  fault_side/1 -> left fault 1 in/2, right fault 1 in/2, left fault 2 in/2, right fault 2 in/2, left fault 3 in/2, right fault 3 in/2
  left fault 1 in/1 -> left fault 1/1
  right fault 1 in/1 -> right fault 1/1
  left fault 2 in/1 -> left fault 2/1
  right fault 2 in/1 -> right fault 2/1
  left fault 3 in/1 -> left fault 3/1
  right fault 3 in/1 -> right fault 3/1
  mission time(k-1)/1 -> mission time in/2
  mission time in/1 -> mission time/1
  mission time/1 -> mission time(k-1)/1, t_mission out/1
  after done(k-1)/1 -> after done in/1
  after done in/1 -> after done/1
  after done/1 -> after done(k-1)/1, end of run/1
  end of run/1 -> Stop/1
  wL_ref/1 -> wL_ref out/1
  TL_L/1 -> TL_L out/1
  J_extra/1 -> J_L out/1, J_R out/1
  left fault 1/1 -> fs_L out/1
  left fault 2/1 -> fc_L out/1
  left fault 3/1 -> fo_L out/1
  wR_ref/1 -> wR_ref out/1
  TL_R/1 -> TL_R out/1
  right fault 1/1 -> fs_R out/1
  right fault 2/1 -> fc_R out/1
  right fault 3/1 -> fo_R out/1
  E_Wh/1 -> E_Wh out/1

== system AGV_IFOC_BLOCKS/Left wheel drive ==
  w_ref : Inport
  TL : Inport  Port=2
  J_extra : Inport  Port=3
  f_speed_inj : Inport  Port=4
  f_cur_inj : Inport  Port=5
  f_open_inj : Inport  Port=6
  flux_sel : Inport  Port=7
  lut_sel : Inport  Port=8
  speed_mode : Inport  Port=9
  Controller : Subsystem
  Controller out 10 not used : Terminator
  Controller out 5 not used : Terminator
  Controller out 6 not used : Terminator
  Controller out 7 not used : Terminator
  Controller out 8 not used : Terminator
  Controller out 9 not used : Terminator
  Input energy : Integrator
  Inverter and motor : Subsystem
  Plant out 1 not used : Terminator
  Plant out 10 not used : Terminator
  Plant out 11 not used : Terminator
  Plant out 12 not used : Terminator
  Plant out 13 not used : Terminator
  Plant out 14 not used : Terminator
  Plant out 15 not used : Terminator
  Plant out 16 not used : Terminator
  Plant out 2 not used : Terminator
  Plant out 3 not used : Terminator
  Plant out 5 not used : Terminator
  Plant out 6 not used : Terminator
  Plant out 8 not used : Terminator
  Plant out 9 not used : Terminator
  w out : Outport
  E_in out : Outport  Port=2
  f_speed out : Outport  Port=3
  f_cur out : Outport  Port=4
  f_open out : Outport  Port=5
  neutral out : Outport  Port=6
  wires:
  Inverter and motor/17(ia_m out) -> Controller/1(ia_m)
  Inverter and motor/18(ib_m out) -> Controller/2(ib_m)
  Inverter and motor/19(ic_m out) -> Controller/3(ic_m)
  Inverter and motor/20(w_m out) -> Controller/4(w_m)
  w_ref/1 -> Controller/5(w_ref)
  flux_sel/1 -> Controller/6(flux_sel)
  lut_sel/1 -> Controller/7(lut_sel)
  speed_mode/1 -> Controller/8(speed_mode)
  Controller/1(da out) -> Inverter and motor/1(da)
  Controller/2(db out) -> Inverter and motor/2(db)
  Controller/3(dc out) -> Inverter and motor/3(dc)
  Controller/4(neutral out) -> Inverter and motor/4(neutral), neutral out/1
  TL/1 -> Inverter and motor/5(TL)
  J_extra/1 -> Inverter and motor/6(J_extra)
  f_speed_inj/1 -> Inverter and motor/7(f_speed)
  f_cur_inj/1 -> Inverter and motor/8(f_cur)
  f_open_inj/1 -> Inverter and motor/9(f_open)
  Inverter and motor/7(P_in out) -> Input energy/1
  Inverter and motor/4(w out) -> w out/1
  Input energy/1 -> E_in out/1
  Controller/11(f_speed out) -> f_speed out/1
  Controller/12(f_cur out) -> f_cur out/1
  Controller/13(f_open out) -> f_open out/1
  Controller/5(w_u out) -> Controller out 5 not used/1
  Controller/6(w_est out) -> Controller out 6 not used/1
  Controller/7(Te_ref out) -> Controller out 7 not used/1
  Controller/8(psi_ref out) -> Controller out 8 not used/1
  Controller/9(psi_est out) -> Controller out 9 not used/1
  Controller/10(Te_est out) -> Controller out 10 not used/1
  Inverter and motor/1(ia out) -> Plant out 1 not used/1
  Inverter and motor/2(ib out) -> Plant out 2 not used/1
  Inverter and motor/3(ic out) -> Plant out 3 not used/1
  Inverter and motor/5(Te out) -> Plant out 5 not used/1
  Inverter and motor/6(psir_mag out) -> Plant out 6 not used/1
  Inverter and motor/8(Pel out) -> Plant out 8 not used/1
  Inverter and motor/9(Pcond out) -> Plant out 9 not used/1
  Inverter and motor/10(Psw out) -> Plant out 10 not used/1
  Inverter and motor/11(Pfe out) -> Plant out 11 not used/1
  Inverter and motor/12(Pout out) -> Plant out 12 not used/1
  Inverter and motor/13(Pfric out) -> Plant out 13 not used/1
  Inverter and motor/14(transitions out) -> Plant out 14 not used/1
  Inverter and motor/15(psim_mag out) -> Plant out 15 not used/1
  Inverter and motor/16(mode out) -> Plant out 16 not used/1

== system AGV_IFOC_BLOCKS/Right wheel drive ==
  w_ref : Inport
  TL : Inport  Port=2
  J_extra : Inport  Port=3
  f_speed_inj : Inport  Port=4
  f_cur_inj : Inport  Port=5
  f_open_inj : Inport  Port=6
  flux_sel : Inport  Port=7
  lut_sel : Inport  Port=8
  speed_mode : Inport  Port=9
  Controller : Subsystem
  Controller out 10 not used : Terminator
  Controller out 5 not used : Terminator
  Controller out 6 not used : Terminator
  Controller out 7 not used : Terminator
  Controller out 8 not used : Terminator
  Controller out 9 not used : Terminator
  Input energy : Integrator
  Inverter and motor : Subsystem
  Plant out 1 not used : Terminator
  Plant out 10 not used : Terminator
  Plant out 11 not used : Terminator
  Plant out 12 not used : Terminator
  Plant out 13 not used : Terminator
  Plant out 14 not used : Terminator
  Plant out 15 not used : Terminator
  Plant out 16 not used : Terminator
  Plant out 2 not used : Terminator
  Plant out 3 not used : Terminator
  Plant out 5 not used : Terminator
  Plant out 6 not used : Terminator
  Plant out 8 not used : Terminator
  Plant out 9 not used : Terminator
  w out : Outport
  E_in out : Outport  Port=2
  f_speed out : Outport  Port=3
  f_cur out : Outport  Port=4
  f_open out : Outport  Port=5
  neutral out : Outport  Port=6
  wires:
  Inverter and motor/17(ia_m out) -> Controller/1(ia_m)
  Inverter and motor/18(ib_m out) -> Controller/2(ib_m)
  Inverter and motor/19(ic_m out) -> Controller/3(ic_m)
  Inverter and motor/20(w_m out) -> Controller/4(w_m)
  w_ref/1 -> Controller/5(w_ref)
  flux_sel/1 -> Controller/6(flux_sel)
  lut_sel/1 -> Controller/7(lut_sel)
  speed_mode/1 -> Controller/8(speed_mode)
  Controller/1(da out) -> Inverter and motor/1(da)
  Controller/2(db out) -> Inverter and motor/2(db)
  Controller/3(dc out) -> Inverter and motor/3(dc)
  Controller/4(neutral out) -> Inverter and motor/4(neutral), neutral out/1
  TL/1 -> Inverter and motor/5(TL)
  J_extra/1 -> Inverter and motor/6(J_extra)
  f_speed_inj/1 -> Inverter and motor/7(f_speed)
  f_cur_inj/1 -> Inverter and motor/8(f_cur)
  f_open_inj/1 -> Inverter and motor/9(f_open)
  Inverter and motor/7(P_in out) -> Input energy/1
  Inverter and motor/4(w out) -> w out/1
  Input energy/1 -> E_in out/1
  Controller/11(f_speed out) -> f_speed out/1
  Controller/12(f_cur out) -> f_cur out/1
  Controller/13(f_open out) -> f_open out/1
  Controller/5(w_u out) -> Controller out 5 not used/1
  Controller/6(w_est out) -> Controller out 6 not used/1
  Controller/7(Te_ref out) -> Controller out 7 not used/1
  Controller/8(psi_ref out) -> Controller out 8 not used/1
  Controller/9(psi_est out) -> Controller out 9 not used/1
  Controller/10(Te_est out) -> Controller out 10 not used/1
  Inverter and motor/1(ia out) -> Plant out 1 not used/1
  Inverter and motor/2(ib out) -> Plant out 2 not used/1
  Inverter and motor/3(ic out) -> Plant out 3 not used/1
  Inverter and motor/5(Te out) -> Plant out 5 not used/1
  Inverter and motor/6(psir_mag out) -> Plant out 6 not used/1
  Inverter and motor/8(Pel out) -> Plant out 8 not used/1
  Inverter and motor/9(Pcond out) -> Plant out 9 not used/1
  Inverter and motor/10(Psw out) -> Plant out 10 not used/1
  Inverter and motor/11(Pfe out) -> Plant out 11 not used/1
  Inverter and motor/12(Pout out) -> Plant out 12 not used/1
  Inverter and motor/13(Pfric out) -> Plant out 13 not used/1
  Inverter and motor/14(transitions out) -> Plant out 14 not used/1
  Inverter and motor/15(psim_mag out) -> Plant out 15 not used/1
  Inverter and motor/16(mode out) -> Plant out 16 not used/1

== system AGV_IFOC_BLOCKS/Left wheel drive/Controller ==
  ia_m : Inport
  ib_m : Inport  Port=2
  ic_m : Inport  Port=3
  w_m : Inport  Port=4
  w_ref : Inport  Port=5
  flux_sel : Inport  Port=6
  lut_sel : Inport  Port=7
  speed_mode : Inport  Port=8
  Applied voltage and current observer : Subsystem
  Current reconstruction : Subsystem
  Fault detection and isolation : Subsystem
  Flux reference : Subsystem
  IFOC current control and SVPWM : Subsystem
  MRAS speed estimator : Subsystem
  Model inductances : Subsystem
  Speed controller : Subsystem
  Te_est not used in IFOC : Constant  Value=0
  ia_m sample : ZeroOrderHold  SampleTime=Ts
  ib_m sample : ZeroOrderHold  SampleTime=Ts
  ic_m sample : ZeroOrderHold  SampleTime=Ts
  w_m sample : ZeroOrderHold  SampleTime=Ts
  w_ref sample : ZeroOrderHold  SampleTime=Ts
  da out : Outport
  db out : Outport  Port=2
  dc out : Outport  Port=3
  neutral out : Outport  Port=4
  w_u out : Outport  Port=5
  w_est out : Outport  Port=6
  Te_ref out : Outport  Port=7
  psi_ref out : Outport  Port=8
  psi_est out : Outport  Port=9
  Te_est out : Outport  Port=10
  f_speed out : Outport  Port=11
  f_cur out : Outport  Port=12
  f_open out : Outport  Port=13
  wires:
  ia_m/1 -> ia_m sample/1
  ib_m/1 -> ib_m sample/1
  ic_m/1 -> ic_m sample/1
  w_m/1 -> w_m sample/1
  w_ref/1 -> w_ref sample/1
  Flux reference/3(psi_ref_p out) -> Model inductances/1(psi_ref_p)
  ia_m sample/1 -> Current reconstruction/1(ia_m), Fault detection and isolation/2(ia_m)
  ib_m sample/1 -> Current reconstruction/2(ib_m), Fault detection and isolation/3(ib_m), Applied voltage and current observer/4(ib_m)
  ic_m sample/1 -> Current reconstruction/3(ic_m), Fault detection and isolation/4(ic_m)
  Fault detection and isolation/8(f_cur_p out) -> Current reconstruction/4(f_cur_p)
  Fault detection and isolation/9(neutral_p out) -> Current reconstruction/5(neutral_p)
  Applied voltage and current observer/3(obs1_p out) -> Current reconstruction/6(obs1_p)
  Applied voltage and current observer/4(obs3_p out) -> Current reconstruction/7(obs3_p)
  Model inductances/1(Lm_c out) -> Current reconstruction/8(Lm_c), MRAS speed estimator/7(Lm_c), IFOC current control and SVPWM/8(Lm_c), Applied voltage and current observer/6(Lm_c)
  Model inductances/3(Lr_c out) -> Current reconstruction/9(Lr_c), MRAS speed estimator/8(Lr_c), IFOC current control and SVPWM/9(Lr_c), Applied voltage and current observer/8(Lr_c)
  Model inductances/6(D_c out) -> Current reconstruction/10(D_c), Applied voltage and current observer/9(D_c)
  Current reconstruction/1(i_alpha out) -> MRAS speed estimator/1(i_alpha), IFOC current control and SVPWM/1(i_alpha)
  Current reconstruction/2(i_beta out) -> MRAS speed estimator/2(i_beta), IFOC current control and SVPWM/2(i_beta)
  Current reconstruction/4(i_alpha_p out) -> MRAS speed estimator/3(i_alpha_p)
  Current reconstruction/5(i_beta_p out) -> MRAS speed estimator/4(i_beta_p)
  Applied voltage and current observer/1(va_app_p out) -> MRAS speed estimator/5(va_app_p)
  Applied voltage and current observer/2(vb_app_p out) -> MRAS speed estimator/6(vb_app_p)
  Model inductances/4(sLs_c out) -> MRAS speed estimator/9(sLs_c), IFOC current control and SVPWM/10(sLs_c)
  Model inductances/5(tr_c out) -> MRAS speed estimator/10(tr_c), IFOC current control and SVPWM/11(tr_c)
  w_ref sample/1 -> MRAS speed estimator/11(w_ref), Fault detection and isolation/5(w_ref), Speed controller/1(w_ref)
  w_m sample/1 -> MRAS speed estimator/12(w_m), Fault detection and isolation/1(w_m)
  Fault detection and isolation/7(f_speed_p out) -> MRAS speed estimator/13(f_speed_p)
  Flux reference/4(trans_t_p out) -> MRAS speed estimator/14(trans_t_p)
  Flux reference/5(dpsi_rate_p out) -> MRAS speed estimator/15(dpsi_p)
  Speed controller/3(Te_ref_p out) -> MRAS speed estimator/16(Te_ref_p)
  Fault detection and isolation/10(Te_lim_p out) -> MRAS speed estimator/17(Te_lim_p)
  MRAS speed estimator/1(w_est out) -> Fault detection and isolation/6(w_est), w_est out/1
  MRAS speed estimator/2(mras_ok out) -> Fault detection and isolation/7(mras_ok)
  Current reconstruction/3(ia_hat out) -> Fault detection and isolation/8(ia_hat)
  Fault detection and isolation/6(w_u out) -> Speed controller/2(w_u), Flux reference/3(w_u), IFOC current control and SVPWM/6(w_u), Applied voltage and current observer/5(w_u), w_u out/1
  Fault detection and isolation/5(Te_lim out) -> Speed controller/3(Te_lim)
  speed_mode/1 -> Speed controller/4(mode)
  Speed controller/2(e_w out) -> Flux reference/1(e_w)
  Speed controller/1(Te_ref out) -> Flux reference/2(Te_ref), IFOC current control and SVPWM/5(Te_ref), Te_ref out/1
  flux_sel/1 -> Flux reference/4(flux_sel)
  lut_sel/1 -> Flux reference/5(lut_sel)
  Flux reference/1(psi_ref out) -> IFOC current control and SVPWM/3(psi_ref), psi_ref out/1
  Flux reference/2(dpsi_rate out) -> IFOC current control and SVPWM/4(dpsi_rate)
  Fault detection and isolation/4(neutral out) -> IFOC current control and SVPWM/7(neutral), neutral out/1
  Te_est not used in IFOC/1 -> Te_est out/1
  IFOC current control and SVPWM/1(da out) -> Applied voltage and current observer/1(da), da out/1
  IFOC current control and SVPWM/2(db out) -> Applied voltage and current observer/2(db), db out/1
  IFOC current control and SVPWM/3(dc out) -> Applied voltage and current observer/3(dc), dc out/1
  Model inductances/2(Ls_c out) -> Applied voltage and current observer/7(Ls_c)
  IFOC current control and SVPWM/4(psir_est out) -> psi_est out/1
  Fault detection and isolation/1(f_speed out) -> f_speed out/1
  Fault detection and isolation/2(f_cur out) -> f_cur out/1
  Fault detection and isolation/3(f_open out) -> f_open out/1

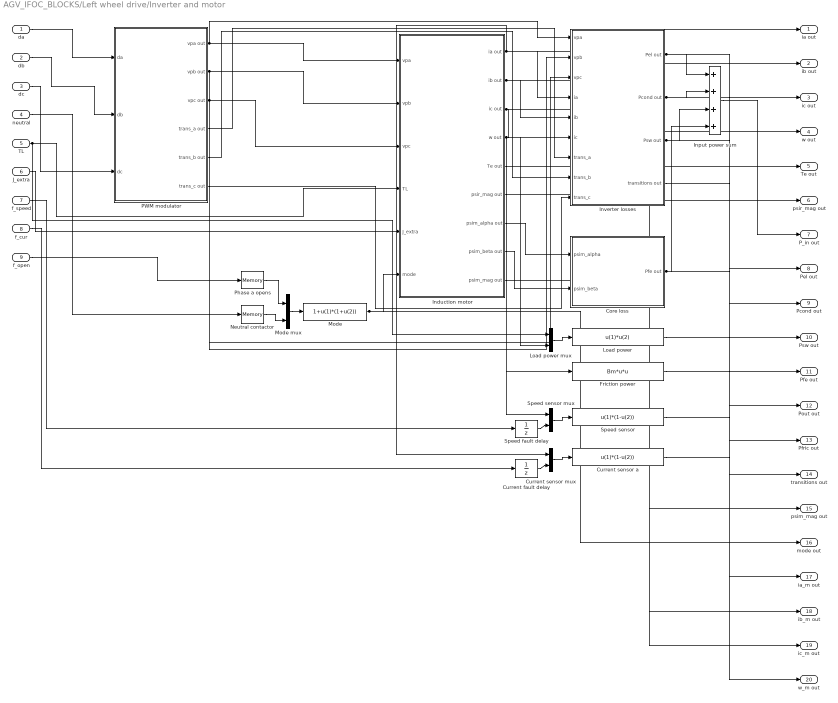
== system AGV_IFOC_BLOCKS/Left wheel drive/Inverter and motor ==
  da : Inport
  db : Inport  Port=2
  dc : Inport  Port=3
  neutral : Inport  Port=4
  TL : Inport  Port=5
  J_extra : Inport  Port=6
  f_speed : Inport  Port=7
  f_cur : Inport  Port=8
  f_open : Inport  Port=9
  Core loss : Subsystem
  Current fault delay : UnitDelay  SampleTime=Ts  HasFrameUpgradeWarning=on
  Current sensor a : Fcn  Expr=u(1)*(1-u(2))
  Current sensor mux : Mux  Inputs=2
  Friction power : Fcn  Expr=Bm*u*u
  Induction motor : Subsystem
  Input power sum : Sum  Inputs=++++
  Inverter losses : Subsystem
  Load power : Fcn  Expr=u(1)*u(2)
  Load power mux : Mux  Inputs=2
  Mode : Fcn  Expr=1+u(1)*(1+u(2))
  Mode mux : Mux  Inputs=2
  Neutral contactor : Memory
  PWM modulator : Subsystem
  Phase a opens : Memory
  Speed fault delay : UnitDelay  SampleTime=Ts  HasFrameUpgradeWarning=on
  Speed sensor : Fcn  Expr=u(1)*(1-u(2))
  Speed sensor mux : Mux  Inputs=2
  ia out : Outport
  ib out : Outport  Port=2
  ic out : Outport  Port=3
  w out : Outport  Port=4
  Te out : Outport  Port=5
  psir_mag out : Outport  Port=6
  P_in out : Outport  Port=7
  Pel out : Outport  Port=8
  Pcond out : Outport  Port=9
  Psw out : Outport  Port=10
  Pfe out : Outport  Port=11
  Pout out : Outport  Port=12
  Pfric out : Outport  Port=13
  transitions out : Outport  Port=14
  psim_mag out : Outport  Port=15
  mode out : Outport  Port=16
  ia_m out : Outport  Port=17
  ib_m out : Outport  Port=18
  ic_m out : Outport  Port=19
  w_m out : Outport  Port=20
  wires:
  neutral/1 -> Neutral contactor/1
  f_open/1 -> Phase a opens/1
  Phase a opens/1 -> Mode mux/1
  Neutral contactor/1 -> Mode mux/2
  Mode mux/1 -> Mode/1
  da/1 -> PWM modulator/1(da)
  db/1 -> PWM modulator/2(db)
  dc/1 -> PWM modulator/3(dc)
  PWM modulator/1(vpa out) -> Induction motor/1(vpa), Inverter losses/1(vpa)
  PWM modulator/2(vpb out) -> Induction motor/2(vpb), Inverter losses/2(vpb)
  PWM modulator/3(vpc out) -> Induction motor/3(vpc), Inverter losses/3(vpc)
  TL/1 -> Induction motor/4(TL), Load power mux/1
  J_extra/1 -> Induction motor/5(J_extra)
  Mode/1 -> Induction motor/6(mode), mode out/1
  Induction motor/1(ia out) -> Inverter losses/4(ia), Current sensor mux/1, ia out/1
  PWM modulator/4(trans_a out) -> Inverter losses/7(trans_a)
  Induction motor/2(ib out) -> Inverter losses/5(ib), ib out/1, ib_m out/1
  PWM modulator/5(trans_b out) -> Inverter losses/8(trans_b)
  Induction motor/3(ic out) -> Inverter losses/6(ic), ic out/1, ic_m out/1
  PWM modulator/6(trans_c out) -> Inverter losses/9(trans_c)
  Induction motor/7(psim_alpha out) -> Core loss/1(psim_alpha)
  Induction motor/8(psim_beta out) -> Core loss/2(psim_beta)
  Induction motor/4(w out) -> Load power mux/2, Friction power/1, Speed sensor mux/1, w out/1
  Load power mux/1 -> Load power/1
  Inverter losses/1(Pel out) -> Input power sum/1, Pel out/1
  Inverter losses/2(Pcond out) -> Input power sum/2, Pcond out/1
  Inverter losses/3(Psw out) -> Input power sum/3, Psw out/1
  Core loss/1(Pfe out) -> Input power sum/4, Pfe out/1
  f_speed/1 -> Speed fault delay/1
  f_cur/1 -> Current fault delay/1
  Speed fault delay/1 -> Speed sensor mux/2
  Speed sensor mux/1 -> Speed sensor/1
  Current fault delay/1 -> Current sensor mux/2
  Current sensor mux/1 -> Current sensor a/1
  Induction motor/5(Te out) -> Te out/1
  Induction motor/6(psir_mag out) -> psir_mag out/1
  Input power sum/1 -> P_in out/1
  Load power/1 -> Pout out/1
  Friction power/1 -> Pfric out/1
  Inverter losses/4(transitions out) -> transitions out/1
  Induction motor/9(psim_mag out) -> psim_mag out/1
  Current sensor a/1 -> ia_m out/1
  Speed sensor/1 -> w_m out/1
